simulink model "chaine_rrc"  (R2023b)
settings: Solver=FixedStepDiscrete  StartTime=0.0  StopTime=2010  FixedStep=Te  RelTol=1e-3
values from neighbouring files (symbols this model uses):
  graine = P.graine    [parametres.m]    (also in parametres_perso.m = mod(sum(c .* (1:numel(c)) * 31) + 7 * numel(c), 2^31 - 1); partie2_1.m)
  N0 = Es / (2*g)    (= 0.158113883008)    [creer_qpsk.m]    (also in creer_qpsk_hamming.m = 0.276699295265; parametres.m = Eb / 10^(EbN0dB/10))
  Te = 1/Lq    [lancer.m]    (also in lancer_echo.m; parametres.m = Tb / L)
undefined symbols (not defined in the file or in its folder): hcoef
settings Model: Creator=e2507477  LastModifiedBy=e2507477

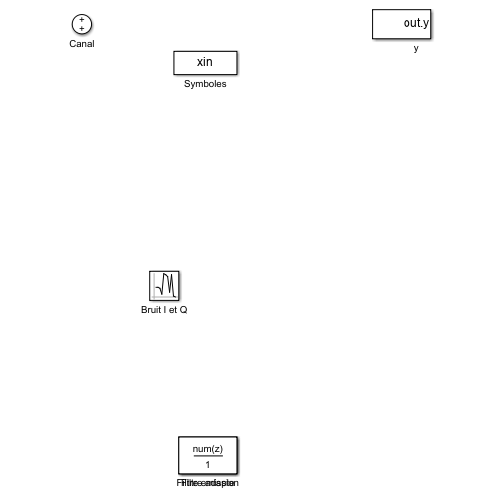
[thumbnail: Simulink's stored preview of the top-level diagram]
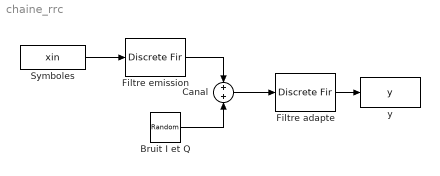
== system chaine_rrc ==
  Bruit I et Q : RandomNumber  Mean=[0 0]  Variance=N0/2*[1 1]  Seed=round(graine) + [50000 90000]  SampleTime=Te
  Canal : Sum
  Filtre adapte : DiscreteFir  Coefficients=hcoef
  Filtre emission : DiscreteFir  Coefficients=hcoef
  Symboles : FromWorkspace  VariableName=xin  SampleTime=Te  Interpolate=off  OutputAfterFinalValue=Holding final value
  y : ToWorkspace  VariableName=y  SampleTime=-1
  wires:
  Symboles/1 -> Filtre emission/1
  Bruit I et Q/1 -> Canal/2
  Filtre emission/1 -> Canal/1
  Filtre adapte/1 -> y/1
  Canal/1 -> Filtre adapte/1
